simulink model "sm_wheel_loader_linkage"  (R2025a)
settings: Solver=ode23t  StartTime=0.0  StopTime=stopTime  RelTol=1e-3  AbsTol=1e-3  EnableMultiTasking=on
PostLoadFcn:
  | set_param([bdroot '/Actuators'],'LabelModeActiveChoice','Ideal')
  | set_param([bdroot '/Linkage'],'popup_actuator_model','Position')
  | 
  | set_param([bdroot '/Actuator Inputs'],'popup_impl','Bucket')
  | set_param([bdroot '/Linkage'],'popup_impl','Bucket')
  | set_param([bdroot '/Load'],'LabelModeActiveChoice','Inertia')
  | set_param([bdroot '/Actuators'],'popup_impl','Bucket')
  | testInput.Active = testInput.BucketYCycle;
StartFcn:
  | tic
StopFcn:
  | Elapsed_Sim_Time = toc;
  | disp(['Elapsed Sim Time = ' num2str(Elapsed_Sim_Time)]);
undefined symbols (not defined in the file or in its folder): X, Y, Z
libraries: sm_lib x10, fl_lib x6, sm_wheel_loader_lib x5, nesl_utility x2, wheel_loader_contact_lib x2, simulink x1
Description:
  | Copyright 2023-2025 The MathWorks, Inc.
settings Model: Creator=smiller  LastModifiedBy=smiller
settings SolverCC: AutoScaleAbsTol=off  AlgebraicLoopSolver=TrustRegion  MaxZcPerStep=1.0
settings DataIOCC: LimitDataPoints=on  MaxDataPoints=10000  ReturnWorkspaceOutputs=off  SignalLoggingName=logsout_sm_wheel_loader_linkage
settings OptimizationCC: ReuseModelBlockBuffer=off  LifeSpan=inf
settings DebuggingCC: UnconnectedInputMsg=warning  UnconnectedOutputMsg=warning  UnconnectedLineMsg=warning  AllowSymbolicDim=off  SubsystemReferenceDiagnosticForUnitTest=warning  SFUnexpectedBacktrackingDiag=warning  SFNoUnconditionalDefaultTransitionDiag=warning  SFExecutionAtInitializationDiag=none  ArithmeticOperatorsInVariantConditions=warning
settings ModelReferenceCC: EnableRefExpFcnMdlSchedulingChecks=on
settings SFSimCC: SimUseLocalCustomCode=off  CustomCodeUndefinedFunction=UseInterfaceOnly
settings RTWCC: RTWUseLocalCustomCode=off  GPUComputeCapability=3.5  DLArmComputeVersion=19.05
settings CodeAppCC: StateflowObjectComments=on
settings GRTTargetCC: TargetLangStandard=C89/C90 (ANSI)
settings ConfigComp: CovMetricSettings=dw  CovSaveCumulativeToWorkspaceVar=on  CovSaveSingleToWorkspaceVar=on  CovExternalEMLEnable=off  CovSFcnEnable=off
settings SimscapeCC: SimscapeLogType=all  SimscapeLogSimulationStatistics=on  SimscapeLogName=simlog_sm_wheel_loader_linkage  SimscapeLogLimitData=off  SimscapeLogDataHistory=10000.0
settings DiagnosticsConfigSet: SimMechanicsConflictingReferenceFrames=none
settings ExplorerConfigSet: InternalSimMechanicsExplorerSettings="<ExplorerConfiguration><canonicalview>default</canonicalview><AnimationSetting><BasePlaybackSpeed>1.0</BasePlaybackSpeed><PlaybackSpeedFactor>4.0</PlaybackSpeedFactor></AnimationSetting><TilePanel><TileInfo><Tiles Columns=\"1\" Count=\"1\" Rows=\"1\"><Column Weight=\"1\"/><Row Weight=\"1\"/><Tile Height=\"1\" Width=\"1\" X=\"0\" Y=\"0\"/></Tiles></TileInfo><SceneInfo><SceneViewer><BGColor><R>1</R><G>1</G><B>1</B></BGColor><Camera><DoPerspective>off</DoPerspective><Position><X>-9.68504522716562377</X><Y>-5.34718256997492336</Y><Z>2.16244753305832393</Z></Position><Center><X>0.176664305406650596</X><Y>-3.69138120840252615</Y><Z>1.55143160632583954</Z></Center><Up><X>0.0627878143914257225</X><Y>-0.0056738157492516629</Y><Z>0.998010770572538064</Z></Up><ViewLimDist>1</ViewLimDist><YLim>1.82950561013908586</YLim><XLim>3.87152954872867205</XLim></Camera></SceneViewer></SceneInfo></TilePanel><MechEditorPanel><Cameras/><GfxPanelCameraMap/><VideoCreator><PlaybackSpeedRatio>1.0</PlaybackSpeedRatio><FrameRate>30</FrameRate><VideoFormat>Motion JPEG AVI</VideoFormat><FrameSize>auto</FrameSize></VideoCreator></MechEditorPanel></ExplorerConfiguration>"

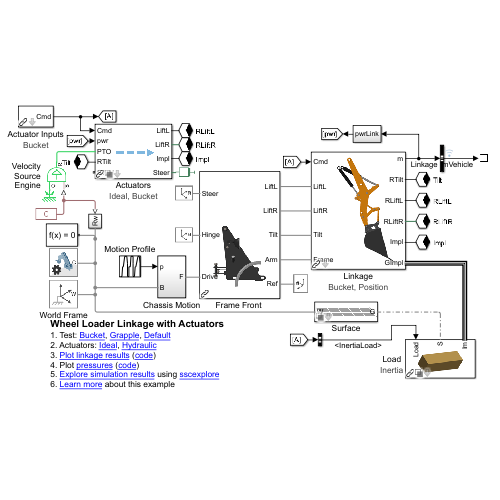
[thumbnail: Simulink's stored preview of the top-level diagram]
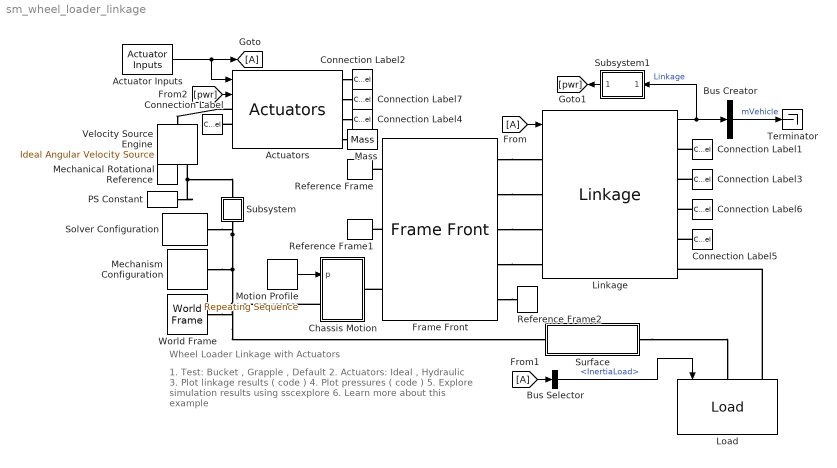
== system sm_wheel_loader_linkage ==
  note: Wheel Loader Linkage with Actuators
  note: 1. Test: Bucket , Grapple , Default
      | 2. Actuators: Ideal , Hydraulic
      | 3. Plot linkage results ( code )
      | 4. Plot pressures ( code )
      | 5. Explore simulation results using sscexplore
      | 6. Learn more about this example
  Actuator Inputs : sm_wheel_loader_lib/Actuator Inputs  popup_steering=off  popup_linkage=on  popup_impl=Bucket
      settings: AttributesFormatString=%<popup_impl>
  Actuators : sm_wheel_loader_lib/Wheel Loader Vehicle/Actuators  VariantControl=Actuators  LabelModeActiveChoice=Ideal  popup_impl=Bucket
      settings: AttributesFormatString=%<LabelModeActiveChoice>, %<popup_impl>
  Bus Creator : BusCreator  Inputs=1
  Bus Selector : BusSelector  OutputSignals=Actuator.InertiaLoad
  Chassis Motion : Subsystem
  Connection Label : ConnectionLabel  Label=Tilt
  Connection Label1 : ConnectionLabel  Label=Tilt
  Connection Label2 : ConnectionLabel  Label=RLiftL
  Connection Label3 : ConnectionLabel  Label=RLiftL
  Connection Label4 : ConnectionLabel  Label=Impl
  Connection Label5 : ConnectionLabel  Label=Impl
  Connection Label6 : ConnectionLabel  Label=RLiftR
  Connection Label7 : ConnectionLabel  Label=RLiftR
  "Frame Front " : sm_wheel_loader_lib/Wheel Loader Vehicle/Frame Front  SystemSampleTime=-1  VariantActivationTime=update diagram  EmptyChoice=off  PassThrough=off  PassThroughVariantControl=(default)  EmptyChoiceVariantControl=(default)  AllowFlexibleInterface=on  Latency=0  AutoFrameSizeCalculation=off
  From : From
  From1 : From
  Goto : Goto
  Linkage : sm_wheel_loader_lib/Wheel Loader Vehicle/Linkage  popup_impl=Bucket  popup_actuator_model=Position
      settings: AttributesFormatString=%<popup_impl>, %<popup_actuator_model>
  Load : sm_wheel_loader_lib/Wheel Loader Vehicle/Load  VariantControl=Choice  LabelModeActiveChoice=Inertia  base_pos=logLoad.LinkTest.basePos  base_ori=logLoad.LinkTest.baseOri  bin_pos=logLoad.LinkTest.binPos  bin_ori=logLoad.LinkTest.binOri
      settings: AttributesFormatString=%<LabelModeActiveChoice>
  Mass : fl_lib/Mechanical/Translational Elements/Mass  mass=1 kg  num_ports=foundation.enum.numPorts2.one  v_specify=off  v_priority=High  v=0 m/s  v_nominal_specify=off  v_nominal_value=1  v_nominal_unit=m/s  f_specify=off  f_priority=None  f=0 N  f_nominal_specify=off  f_nominal_value=1  f_nominal_unit=N
  Mechanical Rotational Reference : fl_lib/Mechanical/Rotational Elements/Mechanical Rotational Reference
  Mechanism Configuration : sm_lib/Utilities/Mechanism Configuration  UniformGravity=Constant  GravityVector=[0 0 -9.80665]  GravityVectorUnits=m/s^2  LinearizationDelta=0.001  JointModeTransitionNonlinearIterations=2
  Motion Profile : simulink/Sources/Repeating Sequence  rep_seq_t=[0 15 20 30 47 65 70]  rep_seq_y=[0 0 1.5 1.5 3 3 2]
  PS Constant : fl_lib/Physical Signals/Sources/PS Constant  constant=HMPST.Eng.wTarget rpm
  Reference Frame : sm_lib/Frames and Transforms/Reference Frame
  Reference Frame1 : sm_lib/Frames and Transforms/Reference Frame
  Reference Frame2 : sm_lib/Frames and Transforms/Reference Frame
  Solver Configuration : nesl_utility/Solver Configuration  PhysicalDomain=network_engine_domain  SubClassName=solver  LeftPortType=input  RightPortType=generic  Tones=[]  Harmonics=[]  SimulateNoise=off  Profile=off  UseLocalSampling=off  EnableSwitchedLinearOptims=on  FrequencyDomain=off  UseCCode=off  RelTol=0.001  AbsTol=0.001  MinStep=1e-09  ToWorkspace=off  RevertToSquareIcSolve=off  NumHomotopyIterations=100  PhasorMode=off  PhasorModeNumHarmonics=1  ConsistencySolver=NEWTON_XTOL_AFTER_FTOL  IndexReductionMethod=DerivativeReplacement  DoDC=off  ResidualTolerance=1e-09  ConsistencyTolSource=GLOBAL  ConsistencyAbsTol=0.001  ConsistencyRelTol=0.001  ConsistencyTolFactor=0.001  UseLocalSolver=off  LocalSolverChoice=NE_BACKWARD_EULER_ADVANCER  ResolveIndetEquations=on  FunctionEvalNumThread=1  LocalSolverSampleTime=0.001  DoFixedCost=off  MaxNonlinIter=3  MaxModeIter=2  ComputeImpulses=off  ImpulseIterations=2  LinearAlgebra=auto  LinearAlgebraNumThread=0  EquationFormulation=NE_TIME_EF  DelaysMemoryBudget=1024  AutomaticFiltering=on  FilteringTimeConstant=0.001  PartitionStorageMethod=AS_NEEDED  PartitionMemoryBudget=1024  PartitionMethod=ROBUST  MultibodyUseLocalSolver=off  MultibodyLocalSolverChoice=ODE1  MultibodyLocalSolverSampleTime=0.001
  Subsystem : Subsystem
  Subsystem1 : Subsystem
  Surface : Subsystem  Variant=on  VariantControlMode=label  VariantControl=Choice  LabelModeActiveChoice=Plane
  Terminator : Terminator
  Velocity Source Engine : fl_lib/Mechanical/Mechanical Sources/Ideal Angular Velocity Source
  World Frame : sm_lib/Frames and Transforms/World Frame
  wires:
  Actuator Inputs/1 -> Actuators/1, Goto/1
  Linkage/1 -> Subsystem1/1(Link), Bus Creator/1  "Linkage"
  Bus Creator/1 -> Terminator/1  "mVehicle"
  From1/1 -> Bus Selector/1
  Bus Selector/1 -> Load/1  "<InertiaLoad>"
  Motion Profile/1 -> Chassis Motion/1(p)
  From/1 -> Linkage/1
  Subsystem1/1(pwr) -> [pwr]
  [pwr] -> Actuators/2
  connections:
  "Frame Front "/LConn1 -- Reference Frame/RConn1
  "Frame Front "/LConn2 -- Reference Frame1/RConn1
  "Frame Front "/RConn5 -- Reference Frame2/RConn1
  Surface/RConn1 -- Load/LConn1
  Solver Configuration/RConn1 -- Subsystem/RConn1 -- Mechanism Configuration/RConn1 -- World Frame/RConn1 -- Surface/LConn1 -- Chassis Motion/LConn1
  "Frame Front "/LConn3 -- Chassis Motion/RConn1
  Load/LConn2 -- Linkage/RConn5
  Actuators/RConn1 -- Connection Label2/LConn1
  Actuators/RConn2 -- Connection Label7/LConn1
  Connection Label1/LConn1 -- Linkage/RConn1
  Connection Label3/LConn1 -- Linkage/RConn2
  Actuators/LConn1 -- Velocity Source Engine/LConn1
  PS Constant/RConn1 -- Subsystem/LConn1 -- Velocity Source Engine/RConn1
  Velocity Source Engine/RConn2 -- Mechanical Rotational Reference/LConn1
  Actuators/RConn4 -- Mass/LConn1
  Connection Label6/LConn1 -- Linkage/RConn3
  "Frame Front "/RConn1 -- Linkage/LConn1
  "Frame Front "/RConn2 -- Linkage/LConn2
  "Frame Front "/RConn3 -- Linkage/LConn3
  "Frame Front "/RConn4 -- Linkage/LConn4
  Actuators/LConn2 -- Connection Label/LConn1
  Actuators/RConn3 -- Connection Label4/LConn1
  Connection Label5/LConn1 -- Linkage/RConn4

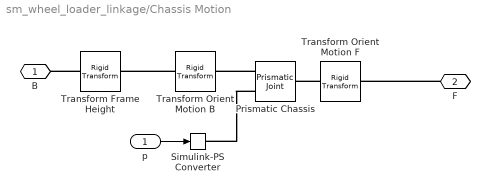
== system sm_wheel_loader_linkage/Chassis Motion ==
  p : Inport
  Prismatic Chassis : sm_lib/Joints/Prismatic Joint  JointMode=Normal  CompositeWrenchDir=FollowerOnBase  CompositeWrenchFrame=BaseFrame  SenseConstraintForce=off  SenseConstraintTorque=off  SenseTotalForce=off  SenseTotalTorque=off  PositionTargetSpecify=off  PositionTargetPriority=High  PositionTargetValue=0  PositionTargetValueUnits=m  VelocityTargetSpecify=off  VelocityTargetPriority=High  VelocityTargetValue=0  VelocityTargetValueUnits=m/s  EquilibriumPosition=0  EquilibriumPositionUnits=m  SpringStiffness=0  SpringStiffnessUnits=N/m  DampingCoefficient=0  DampingCoefficientUnits=N/(m/s)  LowerLimitSpecify=off  LowerLimitBound=-1  LowerLimitBoundUnits=m  LowerLimitStiffness=1e6  LowerLimitStiffnessUnits=N/m  LowerLimitDamping=1e3  LowerLimitDampingUnits=N/(m/s)  LowerLimitTransitionRegionWidth=1e-4  LowerLimitTransitionRegionWidthUnits=m  UpperLimitSpecify=off  UpperLimitBound=1  UpperLimitBoundUnits=m  UpperLimitStiffness=1e6  UpperLimitStiffnessUnits=N/m  UpperLimitDamping=1e3  UpperLimitDampingUnits=N/(m/s)  UpperLimitTransitionRegionWidth=1e-4  UpperLimitTransitionRegionWidthUnits=m  TorqueActuationMode=ComputedTorque  MotionActuationMode=InputMotion  SensePosition=off  SenseVelocity=off  SenseAcceleration=off  SenseTorqueForce=off  SenseLowerLimitTorqueForce=off  SenseUpperLimitTorqueForce=off
  Simulink-PS Converter : nesl_utility/Simulink-PS Converter  PhysicalDomain=network_engine_domain  SubClassName=ps_input  LeftPortType=input  RightPortType=output  PseudoPeriodic=off  Frequencies=[]  NoiseDistribution=none  NoiseParameters=[]  Unit=m  AffineConversion=off  FilteringAndDerivatives=filter  SimscapeFilterOrder=2  InputFilterTimeConstant=0.01  UdotUserProvided=0
  Transform Frame Height : sm_lib/Frames and Transforms/Rigid Transform  RotationMethod=None  FollAlignAxisA=+X  BaseAlignAxisA=+Y  FollAlignAxisB=+Y  BaseAlignAxisB=+Z  RotationStandardAxis=+Z  RotationAngle=0.0  RotationAngleUnits=deg  RotationArbitraryAxis=[0 0 1]  RotationSequenceAxes=FollowerAxes  RotationSequence=XYX  RotationSequenceAngles=[0 0 0]  RotationSequenceAnglesUnits=deg  RotationMatrix=[1 0 0; 0 1 0; 0 0 1]  Quaternion=[1 0 0 0]  TranslationMethod=StandardAxis  TranslationCartesianOffset=[0 0 0]  TranslationCartesianOffsetUnits=m  TranslationStandardAxis=+Z  TranslationStandardOffset=0.65  TranslationStandardOffsetUnits=m  TranslationROffset=0  TranslationROffsetUnits=m  TranslationThetaOffset=0  TranslationThetaOffsetUnits=deg  TranslationZOffset=0  TranslationZOffsetUnits=m
  Transform Orient Motion B : sm_lib/Frames and Transforms/Rigid Transform  RotationMethod=StandardAxis  FollAlignAxisA=+X  BaseAlignAxisA=+Y  FollAlignAxisB=+Y  BaseAlignAxisB=+Z  RotationStandardAxis=+X  RotationAngle=90  RotationAngleUnits=deg  RotationArbitraryAxis=[0 0 1]  RotationSequenceAxes=FollowerAxes  RotationSequence=XYX  RotationSequenceAngles=[0 0 0]  RotationSequenceAnglesUnits=deg  RotationMatrix=[1 0 0; 0 1 0; 0 0 1]  Quaternion=[1 0 0 0]  TranslationMethod=None  TranslationCartesianOffset=[0 0 0]  TranslationCartesianOffsetUnits=m  TranslationStandardAxis=+Z  TranslationStandardOffset=0  TranslationStandardOffsetUnits=m  TranslationROffset=0  TranslationROffsetUnits=m  TranslationThetaOffset=0  TranslationThetaOffsetUnits=deg  TranslationZOffset=0  TranslationZOffsetUnits=m
  Transform Orient Motion F : sm_lib/Frames and Transforms/Rigid Transform  RotationMethod=StandardAxis  FollAlignAxisA=+X  BaseAlignAxisA=+Y  FollAlignAxisB=+Y  BaseAlignAxisB=+Z  RotationStandardAxis=+X  RotationAngle=90  RotationAngleUnits=deg  RotationArbitraryAxis=[0 0 1]  RotationSequenceAxes=FollowerAxes  RotationSequence=XYX  RotationSequenceAngles=[0 0 0]  RotationSequenceAnglesUnits=deg  RotationMatrix=[1 0 0; 0 1 0; 0 0 1]  Quaternion=[1 0 0 0]  TranslationMethod=None  TranslationCartesianOffset=[0 0 0]  TranslationCartesianOffsetUnits=m  TranslationStandardAxis=+Z  TranslationStandardOffset=0  TranslationStandardOffsetUnits=m  TranslationROffset=0  TranslationROffsetUnits=m  TranslationThetaOffset=0  TranslationThetaOffsetUnits=deg  TranslationZOffset=0  TranslationZOffsetUnits=m
  B : PMIOPort  Side=Left
  F : PMIOPort  Port=2  Side=Right
  wires:
  p/1 -> Simulink-PS Converter/1
  connections:
  Prismatic Chassis/LConn2 -- Simulink-PS Converter/RConn1
  Transform Orient Motion F/RConn1 -- Prismatic Chassis/RConn1
  Transform Orient Motion B/LConn1 -- Transform Frame Height/RConn1
  Prismatic Chassis/LConn1 -- Transform Orient Motion B/RConn1
  F/RConn1 -- Transform Orient Motion F/LConn1
  Transform Frame Height/LConn1 -- B/RConn1

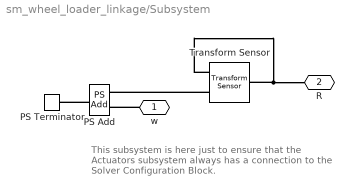
== system sm_wheel_loader_linkage/Subsystem ==
  note: This subsystem is here just to ensure that the Actuators subsystem always has a connection to the Solver Configuration Block.
  PS Add : fl_lib/Physical Signals/Functions/PS Add
  PS Terminator : fl_lib/Physical Signals/Sinks/PS Terminator
  Transform Sensor : sm_lib/Frames and Transforms/Transform Sensor  MeasurementFrame=World  RotationSequence=XYX  SenseAngle=off  SenseAxis=off  SenseQ=off  SenseR=off  SenseRotationSequence=off  SenseOmegaX=off  SenseOmegaY=off  SenseOmegaZ=on  SenseOmega=off  SenseQDot=off  SenseRDot=off  SenseRotationSequenceDot=off  SenseAlphaX=off  SenseAlphaY=off  SenseAlphaZ=off  SenseAlpha=off  SenseQDDot=off  SenseRDDot=off  SenseX=off  SenseY=off  SenseZ=off  SenseXYZ=off  SenseRad=off  SenseAzim=off  SenseDist=off  SenseInc=off  SenseXDot=off  SenseYDot=off  SenseZDot=off  SenseXYZDot=off  SenseRadDot=off  SenseAzimDot=off  SenseDistDot=off  SenseIncDot=off  SenseXDDot=off  SenseYDDot=off  SenseZDDot=off  SenseXYZDDot=off  SenseRadDDot=off  SenseAzimDDot=off  SenseDistDDot=off  SenseIncDDot=off
  w : PMIOPort  Side=Left
  R : PMIOPort  Port=2  Side=Right
  connections:
  Transform Sensor/RConn2 -- PS Add/LConn2
  Transform Sensor/RConn1 -- Transform Sensor/LConn1 -- R/RConn1
  PS Add/RConn1 -- PS Terminator/LConn1
  w/RConn1 -- PS Add/LConn1

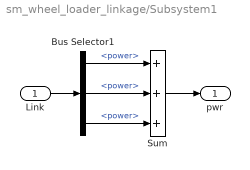
== system sm_wheel_loader_linkage/Subsystem1 ==
  Link : Inport
  Bus Selector1 : BusSelector  OutputSignals=Lift.power,Tilt.power,Impl.power
  Sum : Sum  Inputs=+++
  pwr : Outport
  wires:
  Bus Selector1/1 -> Sum/1  "<power>"
  Link/1 -> Bus Selector1/1
  Bus Selector1/2 -> Sum/2  "<power>"
  Bus Selector1/3 -> Sum/3  "<power>"
  Sum/1 -> pwr/1

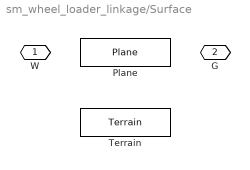
== system sm_wheel_loader_linkage/Surface ==
  Plane : wheel_loader_contact_lib/Plane  VariantControl=Plane
  Terrain : wheel_loader_contact_lib/Terrain  VariantControl=Terrain
  W : PMIOPort  Side=Left
  G : PMIOPort  Port=2  Side=Right
